simulink model "BimanualCarvingModifiedOldEMG"  (R2013a)
settings: Solver=ode4  SolverMode=SingleTasking  StartTime=0.0  StopTime=inf  FixedStep=0.0005  RelTol=1e-3
StartFcn:
  |  warndlg('Dexterit-E models cannot run under simulation. Please compile your model and run it from within Dexterit-E.');set_param(bdroot,'SimulationCommand','stop')
model workspace (MAT data in the model file):
  BKIN_STEP_TIME = 0.0005
  col_x = 1
  col_y = 2
  WIDTH = 3
  HEIGHT = 4
  TARGET_COL = 1
  LOAD = 2
  TRAJ_DURATION_COL = 3
  MAX_LOAD = 2
  FORCE_ON = 1
  HAND_RADIUS = 6
  REST_COL = 4
  TRAINING_COL = 5
  HAND_COLOR = 5
  TARGET_STROKE = 8
  TARGET_RADIUS = 9
  xMaxCursor = 15
  yMaxCursor = 16
  TARGET_COLOR = 7
  START_X = 10
  START_Y = 11
  STIFFNESS_MATERIAL = 3
  MATERIAL_MASS = 4
  MATERIAL_DAMPING = 5
  STIFFNESS_HANDS = 6
  MATERIAL_GOAL_COLOR = 12
  SCALE_VIBRATION = 7
  STONE_WIDTH = 6
  MATERIAL_DUCTILITY = 8
  TARG_COLOR = 1
  TEXT_COLOR = 13
  TEXTBOX_WIDTH = 14
  TEXTBOX_HEIGHT = 15
  ROTATION = 16
  LABEL_TEXT = 17
  LABEL_COLOR = 18
  LABEL_HEIGHT = 19
  ADVANCE_EMG_PLACEMENT = 2
  ADVANCE_EMG_MAX = 3
  EMG_ADVANCE_BUTTON = 1
  EMG_MVC_BUTTON = 2
  START_TRIAL = 3
  END_TRIAL = 4
  MUSC_NUM = 2
  HAND_DISTANCE = 3
  SYN_NUM = 4
undefined symbols (not defined in the file or in its folder): slselsubs
libraries: xpclib x9, simulink x6, General x3, KINARM_loads x2, Video x2, KINARM_IO x1, KINARM_EP_loads x1
(part 5 of 6)

== matlab function BimanualCarvingModifiedOldEMG/Draw_Material/MATLAB Function ==
  data: target input; VCODE output; state_in input; target_type input; opacity_in input; target_display input; x_index input; y_index input; num_states input; stateindices input; target_labels input; KINData input; MaterialPos input; trial_state input
function VCODE = fcn(target, state_in, target_type, opacity_in, target_display, x_index, y_index, num_states, stateindices, target_labels, KINData, MaterialPos, trial_state)

% stateindices should follow this order (depending on target-type):
% 1: fill colour
% 2: stroke colour
% 3: stroke width
% 4: major radius / radius / start point (line)
% 5: minor radius / end point (line)
% 6: orientation angle



% VCODEs are length 70. All units in a VCODE should be SI, e.g. (m) and (rad). Elements in a VCODE are defined as follows:
%
% For all target types:
%  1: target type
%       1 - circle
%       2 - ellipse
%       3 - rectangle
%       4 - line
%       5 - triangle
%       11 - circle with label
%       12 - ellipse with label
%       13 - rectangle with label
%       14 - line with label
%       15 - triangle with label
%  2: target on/off status and target display (which display target will appear on)
%		0 - off
%		1 - on, appearing on both subject and operator displays
%       2 - on, appearing on subject display only
%       3 - on, appearing on operator display only
%  3: x position (m)
%  4: y position (m)
%  5: fill colour (RRGGBB) or texture index
%  6: stroke colour (RRGGBB) or texture index
%  7: stroke width
%  8: reserved for target background ID
%  9: opacity
%
% For circles:
%  10: radius (m)
%
% For ellipses:
%  10: major radius (m)
%  11: minor radius (m)
%  12: orientation of major axis (rad)
%
% For rectangles:
%  10: length (m)
%  11: height (m)
%  12: orientation (rad) (relative to x, y already shown)
%
% For lines:
%  10: endpoint x-axis coordinate relative to start point (m)
%  11: endpoint y-axis coordinate relative to start point (m)
%
% For triangles:
%  10: length (m)
%  11: height (m)
%  12: offset of peak from midpoint of length (m)
%  13: orientation (rad)
%
% For all labelled target types:
%  14: reserved
%  15-64: label characters (indexes in ISO 8859-1 character set)
%  65: label colour (0xRRGGBB), opacity is set by the vcode's opacity (9).
%  66: label height (m)
%  67: reserved
%  68: reserved
%  69: reserved
%  70: reserved

num_targets = size(MaterialPos,2)-1;

% NOTE: we assume that the STATE and/or OPACITY inputs are vectors. 

% If the length of the input STATE is not the same as the number of targets then make STATE a column vector of the same length as 
% the TARGET input, using the first STATE (i.e. all targets get the same state)
if num_targets == length(state_in)
	state = reshape(state_in, num_targets, 1);
else
	state = state_in(1) * ones(num_targets, 1);
end


% If the length of the input OPACITY is not the same as the number of targets then make OPACITY a column vector of the same length as
% the TARGET input, using the first OPACITY (i.e. all targets get the same opacity)
if num_targets == length(opacity_in)
	opacity = reshape(opacity_in, num_targets, 1);
else
	opacity = opacity_in(1) * ones(num_targets, 1);
end


% Clamping the opacity to [0, 100].
opacity = min(opacity, 100);
opacity = max(opacity, 0);

VCODE = zeros(num_targets, 70);

% Set the target type. Targets with labels have type codes 10 greater than their unlabelled counterparts.
VCODE(:, 1) = target_type + 10;
VCODE(:, 2) = target_display;

VCODE(:, 5) = colourshift(target(1, stateindices(state(1), 1)));
VCODE(:, 6) = colourshift(target(1, stateindices(state(1), 1)));

% Set the opacity value
VCODE(:, 9) = opacity_in(1);
% Target only visible during tracking in trial_state==2
%{
if trial_state==0
    VCODE(:, 5) = colourshift(1000000000);
    VCODE(:, 6) = colourshift(1000000000);
    VCODE(:, 9) = 0;
end
%}

% Stroke width
VCODE(:, 7) = target(1, stateindices(state(1), 3))*0.01;

VCODE(:, 3) = MaterialPos(1,1:end-1)';  % x position (m)
VCODE(:, 4) = MaterialPos(2,1:end-1)';  % y position (m)

VCODE(:, 10) = MaterialPos(1,2:end)'-VCODE(:,3);  % line endpoint in x axis, relative to start (m)
VCODE(:, 11) = MaterialPos(2,2:end)'-VCODE(:,4);  % line endpoint in y axis, relative to start (m)

%{
persistent TargetIndex;
if isempty(TargetIndex), TargetIndex = 1; end
% Set the hand position.
if TargetIndex<=length(xMaterial)
    % Initially draw the whole material from left to right
    % Line beginning
    VCODE(:, 3) = xMaterial(TargetIndex);  % x position (m)
    VCODE(:, 4) = yMaterial(TargetIndex);  % y position (m)
    
    % Line endpoint
    VCODE(:, 10) = xMaterial(TargetIndex+1)-VCODE(:,3);  % line endpoint in x axis, relative to start (m)
    VCODE(:, 11) = yMaterial(TargetIndex+1)-VCODE(:,4);  % line endpoint in y axis, relative to start (m)
else
    % After material is all drawn, update only the changing section
    % Line beginning
    VCODE(:, 3) = xMaterial(MaterialUpdateInd1);  % x position (m)
    VCODE(:, 4) = yMaterial(MaterialUpdateInd1);  % y position (m)
    
    % Line endpoint
    VCODE(:, 10) = xMaterial(MaterialUpdateInd2)-VCODE(:,3);  % line endpoint in x axis, relative to start (m)
    VCODE(:, 11) = yMaterial(MaterialUpdateInd2)-VCODE(:,4);  % line endpoint in y axis, relative to start (m)
end


TargetIndex = min(length(xMaterial)+5,TargetIndex+1);
%}
%{
for ii = 1:num_targets
	% Set the target on/off state. If the state input is 0, the target is off. Users of the VCODE should respect this
	% as an indication that the rest of the VCODE will be uninitialized.
	if (state(ii) <= 0) || (state(ii) > num_states)
		VCODE(ii, 2) = 0;  % target is off
	else
		VCODE(ii, 2) = target_display;  % Default is that target is on; target displays as specified by block mask
	end

	fill_colour_col = stateindices(state(ii), 1);
	stroke_colour_col = stateindices(state(ii), 2);
	stroke_width_col = stateindices(state(ii), 3);
	
	% Set the fill colour. Fill colour currently comes from the GUI in RRRGGGBBB format.
	%{
    if fill_colour_col == 0
		VCODE(ii, 5) = -2^31;
	elseif target(fill_colour_col) < 0
		VCODE(ii, 5) = target(ii, fill_colour_col);
	else
		VCODE(ii, 5) = colourshift(target(ii, fill_colour_col));
    end
    %}
    VCODE(ii,5) = colourshift(1000000000);
	
	% Set the stroke colour. Stroke colour currently comes from the GUI in RRRGGGBBB format.
    if trial_state==1
        if stroke_colour_col == 0
            VCODE(ii, 6) = -2^31;
        elseif target(stroke_colour_col) < 0
            VCODE(ii, 6) = target(ii, stroke_colour_col);
        else
            VCODE(ii, 6) = colourshift( target(ii, stroke_colour_col) );
        end
    else
        % CIRCLE APPEARS ONLY DURING TASK
        VCODE(ii, 6) = colourshift(1000000000);
    end

	% Set the stroke width. if target table index for stroke width is zero, then the stroke width is undefined
	if stroke_width_col == 0
		VCODE(ii, 7) = 0;                   % if stroke width column is 0, then stroke width is 0
	elseif stroke_width_col < 0
		VCODE(ii, 7) = 0.001;               % if stroke width column is -ve, then a 1mm default is chosen
	else
		VCODE(ii, 7) = target(ii, stroke_width_col) * 0.01;  % if stroke width column is +ve, convert width from (cm) in target table to (m)
    end

	% Set the opacity value
	VCODE(ii, 9) = opacity(ii);

	% Set attributes specific to each target type. In the process, note the first state vector column used for label information.
	label_index = 1;

	% Set attributes specific to each target type.
	if target_type == 1

		% Handle circle target:
		radius_col = stateindices(state(ii), 4);
		VCODE(ii, 10)=target(ii, radius_col);  % radius (in m)
	    label_index = 5;

	elseif target_type == 2 || target_type == 3

	    % Handle ellipse or rectangle target:
		major_col = stateindices(state(ii), 4);
		minor_col = stateindices(state(ii), 5);
		orientation_col = stateindices(state(ii), 6);
		
		VCODE(ii, 10) = target(ii, major_col) * 0.01;  % major radius (convert from (cm) in target table to (m))
		VCODE(ii, 11) = target(ii, minor_col) * 0.01;  % minor radius (convert from (cm) in target table to (m))
		if orientation_col == 0
			VCODE(ii, 12) = 0;  % if orientation column is 0, set orientation to 0 rad
		else
			VCODE(ii, 12) = mod(target(ii, orientation_col), 360) * pi / 180.0;  % orientation (convert from (degrees) in target table to (rad))
		end
	    label_index = 7;
	
	elseif target_type == 4

		% Handle line target:
		%xendpoint_col = stateindices(state(ii), 4);
		%yendpoint_col = stateindices(state(ii), 5);
		VCODE(ii, 10) = 0;  % line endpoint in x axis, relative to start (m)
		VCODE(ii, 11) = stateindices(state(ii), 1);  % line endpoint in y axis, relative to start (taken from Target Table)
	    label_index = 6;

	elseif target_type == 5

		% Handle triangle target:
		length_col = stateindices(state(ii), 4);
		height_col = stateindices(state(ii), 5);
		offset_col = stateindices(state(ii), 6);
		orientation_col = stateindices(state(ii), 7);

		VCODE(ii, 10) = target(ii, length_col) * 0.01;  % length (convert from (cm) in target table to (m))

		% If the height column is set to 0 then the triangle is automatically made equilateral, with the base length used as length
		% for all sides. If the height column is non-zero, separate values for height and peak offset are taken from the target table.
		if height_col == 0
			VCODE(ii, 11) = sin(pi / 3.0) * VCODE(ii, 10);  % height for equilateral triangle
			VCODE(ii, 12) = 0;                          % peak offset for equilateral triangle
		else
			VCODE(ii, 11) = target(ii, height_col) * 0.01;  % height (convert from (cm) in target table to (m))
			VCODE(ii, 12) = target(ii, offset_col) * 0.01;  % peak offset (convert from (cm) in target table to (m))
		end

		if orientation_col == 0
			VCODE(ii, 13) = 0;  % if orientation column is 0, set orientation to 0 rad
		else
			VCODE(ii, 13) = mod(target(ii, orientation_col), 360) * pi / 180.0;  % orientation (convert from (degrees) in target table to (rad))
		end
	    label_index = 8;
		
	end
	
	% Copy the label characters to the VCODE.
	for jj = 1:50
		VCODE(ii, jj + 14) = target_labels( target( ii, stateindices(state(ii), label_index) ), jj );
	end

	% Set the label colour. Like other colours, label colour comes from the GUI in RRRGGGBBB format and is converted to a 32-bit
	% 0xRRGGBB value here. If the target column table index for the colour is 0, the label is transparent.
	if stateindices(state(ii), label_index + 1) == 0
		VCODE(ii, 65) = -2^31;
	elseif target( ii, stateindices(state(ii), label_index + 1) ) < 0
		VCODE(ii, 65) = target( ii, stateindices(state(ii), label_index + 1) );
	else
		VCODE(ii, 65) = colourshift( target( ii, stateindices(state(ii), label_index + 1) ) );
	end

	% Set the label height. Label height is converted from (cm) in the target table to (m).
	VCODE(ii, 66) = target( ii, stateindices(state, label_index + 2) ) * 0.01;


	
end
%}
% The colourshift function converts an "RRRGGGBBB" colour value to RRGBB (as an uint32).
function RRGGBBAA = colourshift(RRRGGGBBB)

%this is "no fill"
if RRRGGGBBB == 1000000000
    RRGGBBAA = cast(16777216, 'uint32'); %hex 0x1000000
    return; 
end

blue = cast(mod(RRRGGGBBB, 1000), 'uint32');
green = cast(mod(RRRGGGBBB - blue, 1000000) / 1000, 'uint32');
red = cast((RRRGGGBBB - (green * 1000) - blue) / 1000000, 'uint32');

RRGGBBAA = bitshift(red, 16) + bitshift(green, 8) + blue;

== matlab function BimanualCarvingModifiedOldEMG/Draw_Start/MATLAB Function ==
  data: target input; VCODE output; state_in input; target_type input; opacity_in input; target_display input; x_index input; y_index input; num_states input; stateindices input; target_labels input; KINData input; xStart input; yStart input; HandDistance input; trial_state input
function VCODE = fcn(target, state_in, target_type, opacity_in, target_display, x_index, y_index, num_states, stateindices, target_labels, KINData, xStart, yStart, HandDistance, trial_state)

% stateindices should follow this order (depending on target-type):
% 1: fill colour
% 2: stroke colour
% 3: stroke width
% 4: major radius / radius / start point (line)
% 5: minor radius / end point (line)
% 6: orientation angle



% VCODEs are length 70. All units in a VCODE should be SI, e.g. (m) and (rad). Elements in a VCODE are defined as follows:
%
% For all target types:
%  1: target type
%       1 - circle
%       2 - ellipse
%       3 - rectangle
%       4 - line
%       5 - triangle
%       11 - circle with label
%       12 - ellipse with label
%       13 - rectangle with label
%       14 - line with label
%       15 - triangle with label
%  2: target on/off status and target display (which display target will appear on)
%		0 - off
%		1 - on, appearing on both subject and operator displays
%       2 - on, appearing on subject display only
%       3 - on, appearing on operator display only
%  3: x position (m)
%  4: y position (m)
%  5: fill colour (RRGGBB) or texture index
%  6: stroke colour (RRGGBB) or texture index
%  7: stroke width
%  8: reserved for target background ID
%  9: opacity
%
% For circles:
%  10: radius (m)
%
% For ellipses:
%  10: major radius (m)
%  11: minor radius (m)
%  12: orientation of major axis (rad)
%
% For rectangles:
%  10: length (m)
%  11: height (m)
%  12: orientation (rad) (relative to x, y already shown)
%
% For lines:
%  10: endpoint x-axis coordinate relative to start point (m)
%  11: endpoint y-axis coordinate relative to start point (m)
%
% For triangles:
%  10: length (m)
%  11: height (m)
%  12: offset of peak from midpoint of length (m)
%  13: orientation (rad)
%
% For all labelled target types:
%  14: reserved
%  15-64: label characters (indexes in ISO 8859-1 character set)
%  65: label colour (0xRRGGBB), opacity is set by the vcode's opacity (9).
%  66: label height (m)
%  67: reserved
%  68: reserved
%  69: reserved
%  70: reserved

num_targets = 2;

% NOTE: we assume that the STATE and/or OPACITY inputs are vectors. 

% If the length of the input STATE is not the same as the number of targets then make STATE a column vector of the same length as 
% the TARGET input, using the first STATE (i.e. all targets get the same state)
if num_targets == length(state_in)
	state = reshape(state_in, num_targets, 1);
else
	state = state_in(1) * ones(num_targets, 1);
end


% If the length of the input OPACITY is not the same as the number of targets then make OPACITY a column vector of the same length as
% the TARGET input, using the first OPACITY (i.e. all targets get the same opacity)
if num_targets == length(opacity_in)
	opacity = reshape(opacity_in, num_targets, 1);
else
	opacity = opacity_in(1) * ones(num_targets, 1);
end


% Clamping the opacity to [0, 100].
opacity = min(opacity, 100);
opacity = max(opacity, 0);

VCODE = zeros(num_targets, 70);

% Set the target type. Targets with labels have type codes 10 greater than their unlabelled counterparts.
VCODE(:, 1) = target_type + 10;

% Set the hand position.
VCODE(1, 3) = xStart+HandDistance/2;  % x position (m)
VCODE(1, 4) = yStart;  % y position (m)
VCODE(2, 3) = xStart-HandDistance/2;  % x position (m)
VCODE(2, 4) = yStart;  % y position (m)

for ii = 1:num_targets
	% Set the target on/off state. If the state input is 0, the target is off. Users of the VCODE should respect this
	% as an indication that the rest of the VCODE will be uninitialized.
    
	if (state(1) <= 0) || (state(1) > num_states)
		VCODE(ii, 2) = 0;  % target is off
	else
		VCODE(ii, 2) = target_display;  % Default is that target is on; target displays as specified by block mask
    end
    

	fill_colour_col = stateindices(state(1), 1);
	stroke_colour_col = stateindices(state(1), 2);
	stroke_width_col = stateindices(state(1), 3);
	
	% Set the fill colour. Fill colour currently comes from the GUI in RRRGGGBBB format.
	%{
    if fill_colour_col == 0
		VCODE(ii, 5) = -2^31;
	elseif target(fill_colour_col) < 0
		VCODE(ii, 5) = target(ii, fill_colour_col);
	else
		VCODE(ii, 5) = colourshift(target(ii, fill_colour_col));
    end
    %}
    VCODE(ii,5) = colourshift(1000000000);
	
	% Set the stroke colour. Stroke colour currently comes from the GUI in RRRGGGBBB format.
	if stroke_colour_col == 0
		VCODE(ii, 6) = -2^31;
	elseif target(stroke_colour_col) < 0
		VCODE(ii, 6) = target(1, stroke_colour_col);
	else
		VCODE(ii, 6) = colourshift( target(1, stroke_colour_col) );
    end
    if trial_state~=0
        VCODE(ii,5) = colourshift(1000000000);
    end

	% Set the stroke width. if target table index for stroke width is zero, then the stroke width is undefined
	if stroke_width_col == 0
		VCODE(ii, 7) = 0;                   % if stroke width column is 0, then stroke width is 0
	elseif stroke_width_col < 0
		VCODE(ii, 7) = 0.001;               % if stroke width column is -ve, then a 1mm default is chosen
	else
		VCODE(ii, 7) = target(1, stroke_width_col) * 0.01 * 3;  % if stroke width column is +ve, convert width from (cm) in target table to (m)
    end
    if trial_state==1
        VCODE(ii,7) = 0;
    end

	% Set the opacity value
    VCODE(ii, 9) = 100;

	% Set attributes specific to each target type. In the process, note the first state vector column used for label information.
	label_index = 1;

	% Set attributes specific to each target type.
	if target_type == 1

		% Handle circle target:
		radius_col = stateindices(state(1), 4);
		VCODE(ii, 10)=target(1, radius_col);  % radius (in m)
	    label_index = 5;

	elseif target_type == 2 || target_type == 3

	    % Handle ellipse or rectangle target:
		major_col = stateindices(state(ii), 4);
		minor_col = stateindices(state(ii), 5);
		orientation_col = stateindices(state(ii), 6);
		
		VCODE(ii, 10) = target(ii, major_col) * 0.01;  % major radius (convert from (cm) in target table to (m))
		VCODE(ii, 11) = target(ii, minor_col) * 0.01;  % minor radius (convert from (cm) in target table to (m))
		if orientation_col == 0
			VCODE(ii, 12) = 0;  % if orientation column is 0, set orientation to 0 rad
		else
			VCODE(ii, 12) = mod(target(ii, orientation_col), 360) * pi / 180.0;  % orientation (convert from (degrees) in target table to (rad))
		end
	    label_index = 7;
	
	elseif target_type == 4

		% Handle line target:
		%xendpoint_col = stateindices(state(ii), 4);
		%yendpoint_col = stateindices(state(ii), 5);
		VCODE(ii, 10) = 0;  % line endpoint in x axis, relative to start (m)
		VCODE(ii, 11) = stateindices(state(ii), 1);  % line endpoint in y axis, relative to start (taken from Target Table)
	    label_index = 6;

	elseif target_type == 5

		% Handle triangle target:
		length_col = stateindices(state(ii), 4);
		height_col = stateindices(state(ii), 5);
		offset_col = stateindices(state(ii), 6);
		orientation_col = stateindices(state(ii), 7);

		VCODE(ii, 10) = target(ii, length_col) * 0.01;  % length (convert from (cm) in target table to (m))

		% If the height column is set to 0 then the triangle is automatically made equilateral, with the base length used as length
		% for all sides. If the height column is non-zero, separate values for height and peak offset are taken from the target table.
		if height_col == 0
			VCODE(ii, 11) = sin(pi / 3.0) * VCODE(ii, 10);  % height for equilateral triangle
			VCODE(ii, 12) = 0;                          % peak offset for equilateral triangle
		else
			VCODE(ii, 11) = target(ii, height_col) * 0.01;  % height (convert from (cm) in target table to (m))
			VCODE(ii, 12) = target(ii, offset_col) * 0.01;  % peak offset (convert from (cm) in target table to (m))
		end

		if orientation_col == 0
			VCODE(ii, 13) = 0;  % if orientation column is 0, set orientation to 0 rad
		else
			VCODE(ii, 13) = mod(target(ii, orientation_col), 360) * pi / 180.0;  % orientation (convert from (degrees) in target table to (rad))
		end
	    label_index = 8;
		
	end
	%{
	% Copy the label characters to the VCODE.
	for jj = 1:50
		VCODE(ii, jj + 14) = target_labels( target( ii, stateindices(state(ii), label_index) ), jj );
	end

	% Set the label colour. Like other colours, label colour comes from the GUI in RRRGGGBBB format and is converted to a 32-bit
	% 0xRRGGBB value here. If the target column table index for the colour is 0, the label is transparent.
	if stateindices(state(ii), label_index + 1) == 0
		VCODE(ii, 65) = -2^31;
	elseif target( ii, stateindices(state(ii), label_index + 1) ) < 0
		VCODE(ii, 65) = target( ii, stateindices(state(ii), label_index + 1) );
	else
		VCODE(ii, 65) = colourshift( target( ii, stateindices(state(ii), label_index + 1) ) );
	end

	% Set the label height. Label height is converted from (cm) in the target table to (m).
	VCODE(ii, 66) = target( ii, stateindices(state, label_index + 2) ) * 0.01;
    %}

	
end

% The colourshift function converts an "RRRGGGBBB" colour value to RRGBB (as an uint32).
function RRGGBBAA = colourshift(RRRGGGBBB)

%this is "no fill"
if RRRGGGBBB == 1000000000
    RRGGBBAA = cast(16777216, 'uint32'); %hex 0x1000000
    return; 
end

blue = cast(mod(RRRGGGBBB, 1000), 'uint32');
green = cast(mod(RRRGGGBBB - blue, 1000000) / 1000, 'uint32');
red = cast((RRRGGGBBB - (green * 1000) - blue) / 1000000, 'uint32');

RRGGBBAA = bitshift(red, 16) + bitshift(green, 8) + blue;

== matlab function BimanualCarvingModifiedOldEMG/Draw_MaterialTarget/MATLAB Function ==
  data: target input; VCODE output; state_in input; target_type input; opacity_in input; target_display input; x_index input; y_index input; num_states input; stateindices input; target_labels input; KINData input; MaterialPos input; trial_state input
function VCODE = fcn(target, state_in, target_type, opacity_in, target_display, x_index, y_index, num_states, stateindices, target_labels, KINData, MaterialPos, trial_state)

% stateindices should follow this order (depending on target-type):
% 1: fill colour
% 2: stroke colour
% 3: stroke width
% 4: major radius / radius / start point (line)
% 5: minor radius / end point (line)
% 6: orientation angle



% VCODEs are length 70. All units in a VCODE should be SI, e.g. (m) and (rad). Elements in a VCODE are defined as follows:
%
% For all target types:
%  1: target type
%       1 - circle
%       2 - ellipse
%       3 - rectangle
%       4 - line
%       5 - triangle
%       11 - circle with label
%       12 - ellipse with label
%       13 - rectangle with label
%       14 - line with label
%       15 - triangle with label
%  2: target on/off status and target display (which display target will appear on)
%		0 - off
%		1 - on, appearing on both subject and operator displays
%       2 - on, appearing on subject display only
%       3 - on, appearing on operator display only
%  3: x position (m)
%  4: y position (m)
%  5: fill colour (RRGGBB) or texture index
%  6: stroke colour (RRGGBB) or texture index
%  7: stroke width
%  8: reserved for target background ID
%  9: opacity
%
% For circles:
%  10: radius (m)
%
% For ellipses:
%  10: major radius (m)
%  11: minor radius (m)
%  12: orientation of major axis (rad)
%
% For rectangles:
%  10: length (m)
%  11: height (m)
%  12: orientation (rad) (relative to x, y already shown)
%
% For lines:
%  10: endpoint x-axis coordinate relative to start point (m)
%  11: endpoint y-axis coordinate relative to start point (m)
%
% For triangles:
%  10: length (m)
%  11: height (m)
%  12: offset of peak from midpoint of length (m)
%  13: orientation (rad)
%
% For all labelled target types:
%  14: reserved
%  15-64: label characters (indexes in ISO 8859-1 character set)
%  65: label colour (0xRRGGBB), opacity is set by the vcode's opacity (9).
%  66: label height (m)
%  67: reserved
%  68: reserved
%  69: reserved
%  70: reserved

num_targets = size(MaterialPos,2)-1;

% NOTE: we assume that the STATE and/or OPACITY inputs are vectors. 

% If the length of the input STATE is not the same as the number of targets then make STATE a column vector of the same length as 
% the TARGET input, using the first STATE (i.e. all targets get the same state)
if num_targets == length(state_in)
	state = reshape(state_in, num_targets, 1);
else
	state = state_in(1) * ones(num_targets, 1);
end


% If the length of the input OPACITY is not the same as the number of targets then make OPACITY a column vector of the same length as
% the TARGET input, using the first OPACITY (i.e. all targets get the same opacity)
if num_targets == length(opacity_in)
	opacity = reshape(opacity_in, num_targets, 1);
else
	opacity = opacity_in(1) * ones(num_targets, 1);
end


% Clamping the opacity to [0, 100].
opacity = min(opacity, 100);
opacity = max(opacity, 0);

VCODE = zeros(num_targets, 70);

% Set the target type. Targets with labels have type codes 10 greater than their unlabelled counterparts.
VCODE(:, 1) = target_type + 10;
VCODE(:, 2) = target_display;

VCODE(:, 5) = colourshift(target(1, stateindices(state(1), 1)));
VCODE(:, 6) = colourshift(target(1, stateindices(state(1), 1)));

% Set the opacity value
VCODE(:, 9) = opacity_in(1);
% Target only visible during tracking in trial_state==2
%{
if trial_state==0
    VCODE(:, 5) = colourshift(1000000000);
    VCODE(:, 6) = colourshift(1000000000);
    VCODE(:, 9) = 0;
end
%}

% Stroke width
VCODE(:, 7) = target(1, stateindices(state(1), 3))*0.01;

VCODE(:, 3) = MaterialPos(1,1:end-1)';  % x position (m)
VCODE(:, 4) = MaterialPos(2,1:end-1)';  % y position (m)

VCODE(:, 10) = MaterialPos(1,2:end)'-VCODE(:,3);  % line endpoint in x axis, relative to start (m)
VCODE(:, 11) = MaterialPos(2,2:end)'-VCODE(:,4);  % line endpoint in y axis, relative to start (m)

%{
persistent TargetIndex;
if isempty(TargetIndex), TargetIndex = 1; end
% Set the hand position.
if TargetIndex<=length(xMaterial)
    % Initially draw the whole material from left to right
    % Line beginning
    VCODE(:, 3) = xMaterial(TargetIndex);  % x position (m)
    VCODE(:, 4) = yMaterial(TargetIndex);  % y position (m)
    
    % Line endpoint
    VCODE(:, 10) = xMaterial(TargetIndex+1)-VCODE(:,3);  % line endpoint in x axis, relative to start (m)
    VCODE(:, 11) = yMaterial(TargetIndex+1)-VCODE(:,4);  % line endpoint in y axis, relative to start (m)
else
    % After material is all drawn, update only the changing section
    % Line beginning
    VCODE(:, 3) = xMaterial(MaterialUpdateInd1);  % x position (m)
    VCODE(:, 4) = yMaterial(MaterialUpdateInd1);  % y position (m)
    
    % Line endpoint
    VCODE(:, 10) = xMaterial(MaterialUpdateInd2)-VCODE(:,3);  % line endpoint in x axis, relative to start (m)
    VCODE(:, 11) = yMaterial(MaterialUpdateInd2)-VCODE(:,4);  % line endpoint in y axis, relative to start (m)
end


TargetIndex = min(length(xMaterial)+5,TargetIndex+1);
%}
%{
for ii = 1:num_targets
	% Set the target on/off state. If the state input is 0, the target is off. Users of the VCODE should respect this
	% as an indication that the rest of the VCODE will be uninitialized.
	if (state(ii) <= 0) || (state(ii) > num_states)
		VCODE(ii, 2) = 0;  % target is off
	else
		VCODE(ii, 2) = target_display;  % Default is that target is on; target displays as specified by block mask
	end

	fill_colour_col = stateindices(state(ii), 1);
	stroke_colour_col = stateindices(state(ii), 2);
	stroke_width_col = stateindices(state(ii), 3);
	
	% Set the fill colour. Fill colour currently comes from the GUI in RRRGGGBBB format.
	%{
    if fill_colour_col == 0
		VCODE(ii, 5) = -2^31;
	elseif target(fill_colour_col) < 0
		VCODE(ii, 5) = target(ii, fill_colour_col);
	else
		VCODE(ii, 5) = colourshift(target(ii, fill_colour_col));
    end
    %}
    VCODE(ii,5) = colourshift(1000000000);
	
	% Set the stroke colour. Stroke colour currently comes from the GUI in RRRGGGBBB format.
    if trial_state==1
        if stroke_colour_col == 0
            VCODE(ii, 6) = -2^31;
        elseif target(stroke_colour_col) < 0
            VCODE(ii, 6) = target(ii, stroke_colour_col);
        else
            VCODE(ii, 6) = colourshift( target(ii, stroke_colour_col) );
        end
    else
        % CIRCLE APPEARS ONLY DURING TASK
        VCODE(ii, 6) = colourshift(1000000000);
    end

	% Set the stroke width. if target table index for stroke width is zero, then the stroke width is undefined
	if stroke_width_col == 0
		VCODE(ii, 7) = 0;                   % if stroke width column is 0, then stroke width is 0
	elseif stroke_width_col < 0
		VCODE(ii, 7) = 0.001;               % if stroke width column is -ve, then a 1mm default is chosen
	else
		VCODE(ii, 7) = target(ii, stroke_width_col) * 0.01;  % if stroke width column is +ve, convert width from (cm) in target table to (m)
    end

	% Set the opacity value
	VCODE(ii, 9) = opacity(ii);

	% Set attributes specific to each target type. In the process, note the first state vector column used for label information.
	label_index = 1;

	% Set attributes specific to each target type.
	if target_type == 1

		% Handle circle target:
		radius_col = stateindices(state(ii), 4);
		VCODE(ii, 10)=target(ii, radius_col);  % radius (in m)
	    label_index = 5;

	elseif target_type == 2 || target_type == 3

	    % Handle ellipse or rectangle target:
		major_col = stateindices(state(ii), 4);
		minor_col = stateindices(state(ii), 5);
		orientation_col = stateindices(state(ii), 6);
		
		VCODE(ii, 10) = target(ii, major_col) * 0.01;  % major radius (convert from (cm) in target table to (m))
		VCODE(ii, 11) = target(ii, minor_col) * 0.01;  % minor radius (convert from (cm) in target table to (m))
		if orientation_col == 0
			VCODE(ii, 12) = 0;  % if orientation column is 0, set orientation to 0 rad
		else
			VCODE(ii, 12) = mod(target(ii, orientation_col), 360) * pi / 180.0;  % orientation (convert from (degrees) in target table to (rad))
		end
	    label_index = 7;
	
	elseif target_type == 4

		% Handle line target:
		%xendpoint_col = stateindices(state(ii), 4);
		%yendpoint_col = stateindices(state(ii), 5);
		VCODE(ii, 10) = 0;  % line endpoint in x axis, relative to start (m)
		VCODE(ii, 11) = stateindices(state(ii), 1);  % line endpoint in y axis, relative to start (taken from Target Table)
	    label_index = 6;

	elseif target_type == 5

		% Handle triangle target:
		length_col = stateindices(state(ii), 4);
		height_col = stateindices(state(ii), 5);
		offset_col = stateindices(state(ii), 6);
		orientation_col = stateindices(state(ii), 7);

		VCODE(ii, 10) = target(ii, length_col) * 0.01;  % length (convert from (cm) in target table to (m))

		% If the height column is set to 0 then the triangle is automatically made equilateral, with the base length used as length
		% for all sides. If the height column is non-zero, separate values for height and peak offset are taken from the target table.
		if height_col == 0
			VCODE(ii, 11) = sin(pi / 3.0) * VCODE(ii, 10);  % height for equilateral triangle
			VCODE(ii, 12) = 0;                          % peak offset for equilateral triangle
		else
			VCODE(ii, 11) = target(ii, height_col) * 0.01;  % height (convert from (cm) in target table to (m))
			VCODE(ii, 12) = target(ii, offset_col) * 0.01;  % peak offset (convert from (cm) in target table to (m))
		end

		if orientation_col == 0
			VCODE(ii, 13) = 0;  % if orientation column is 0, set orientation to 0 rad
		else
			VCODE(ii, 13) = mod(target(ii, orientation_col), 360) * pi / 180.0;  % orientation (convert from (degrees) in target table to (rad))
		end
	    label_index = 8;
		
	end
	
	% Copy the label characters to the VCODE.
	for jj = 1:50
		VCODE(ii, jj + 14) = target_labels( target( ii, stateindices(state(ii), label_index) ), jj );
	end

	% Set the label colour. Like other colours, label colour comes from the GUI in RRRGGGBBB format and is converted to a 32-bit
	% 0xRRGGBB value here. If the target column table index for the colour is 0, the label is transparent.
	if stateindices(state(ii), label_index + 1) == 0
		VCODE(ii, 65) = -2^31;
	elseif target( ii, stateindices(state(ii), label_index + 1) ) < 0
		VCODE(ii, 65) = target( ii, stateindices(state(ii), label_index + 1) );
	else
		VCODE(ii, 65) = colourshift( target( ii, stateindices(state(ii), label_index + 1) ) );
	end

	% Set the label height. Label height is converted from (cm) in the target table to (m).
	VCODE(ii, 66) = target( ii, stateindices(state, label_index + 2) ) * 0.01;


	
end
%}
% The colourshift function converts an "RRRGGGBBB" colour value to RRGBB (as an uint32).
function RRGGBBAA = colourshift(RRRGGGBBB)

%this is "no fill"
if RRRGGGBBB == 1000000000
    RRGGBBAA = cast(16777216, 'uint32'); %hex 0x1000000
    return; 
end

blue = cast(mod(RRRGGGBBB, 1000), 'uint32');
green = cast(mod(RRRGGGBBB - blue, 1000000) / 1000, 'uint32');
red = cast((RRRGGGBBB - (green * 1000) - blue) / 1000000, 'uint32');

RRGGBBAA = bitshift(red, 16) + bitshift(green, 8) + blue;

== matlab function BimanualCarvingModifiedOldEMG/Parameter_columns/MATLAB Function ==
  data: target input; VCODE output; state_in input; target_type input; opacity_in input; target_display input; x_index input; y_index input; num_states input; stateindices input; target_labels input
function VCODE = fcn(target, state_in, target_type, opacity_in, target_display, x_index, y_index, num_states, stateindices, target_labels)

VCODE = zeros(1,70);
% SIMPLY ASSIGN TOOL LENGTH AND WIDTH TO OUTPUT, NOT REAL VCODE!!
VCODE(1,1) = target(1,stateindices(1,1)); % tool width (m)
VCODE(1,2) = target(1,stateindices(1,2)); % tool length (m)
VCODE(1,3) = target(1,stateindices(1,3)); % frame inner width (m)
VCODE(1,4) = target(1,stateindices(1,4)); % frame outer width (m)
VCODE(1,5) = target(1,stateindices(1,5)); % force on?
VCODE(1,6) = target(1,stateindices(1,6)); % start radius (m)
VCODE(1,7) = target(1,stateindices(1,7)); % end radius (m)
%{
% stateindices should follow this order (depending on target-type):
% 1: fill colour
% 2: stroke colour
% 3: stroke width
% 4: major radius / radius / start point (line)
% 5: minor radius / end point (line)
% 6: orientation angle



% VCODEs are length 70. All units in a VCODE should be SI, e.g. (m) and (rad). Elements in a VCODE are defined as follows:
%
% For all target types:
%  1: target type
%       1 - circle
%       2 - ellipse
%       3 - rectangle
%       4 - line
%       5 - triangle
%       11 - circle with label
%       12 - ellipse with label
%       13 - rectangle with label
%       14 - line with label
%       15 - triangle with label
%  2: target on/off status and target display (which display target will appear on)
%		0 - off
%		1 - on, appearing on both subject and operator displays
%       2 - on, appearing on subject display only
%       3 - on, appearing on operator display only
%  3: x position (m)
%  4: y position (m)
%  5: fill colour (RRGGBB) or texture index
%  6: stroke colour (RRGGBB) or texture index
%  7: stroke width
%  8: reserved for target background ID
%  9: opacity
%
% For circles:
%  10: radius (m)
%
% For ellipses:
%  10: major radius (m)
%  11: minor radius (m)
%  12: orientation of major axis (rad)
%
% For rectangles:
%  10: length (m)
%  11: height (m)
%  12: orientation (rad) (relative to x, y already shown)
%
% For lines:
%  10: endpoint x-axis coordinate relative to start point (m)
%  11: endpoint y-axis coordinate relative to start point (m)
%
% For triangles:
%  10: length (m)
%  11: height (m)
%  12: offset of peak from midpoint of length (m)
%  13: orientation (rad)
%
% For all labelled target types:
%  14: reserved
%  15-64: label characters (indexes in ISO 8859-1 character set)
%  65: label colour (0xRRGGBB), opacity is set by the vcode's opacity (9).
%  66: label height (m)
%  67: reserved
%  68: reserved
%  69: reserved
%  70: reserved

num_targets = size(target, 1);

% NOTE: we assume that the STATE and/or OPACITY inputs are vectors. 

% If the length of the input STATE is not the same as the number of targets then make STATE a column vector of the same length as 
% the TARGET input, using the first STATE (i.e. all targets get the same state) 
if num_targets == length(state_in)
	state = reshape(state_in, num_targets, 1);
else
	state = state_in(1) * ones(num_targets, 1);
end


% If the length of the input OPACITY is not the same as the number of targets then make OPACITY a column vector of the same length as
% the TARGET input, using the first OPACITY (i.e. all targets get the same opacity) 
if num_targets == length(opacity_in)
	opacity = reshape(opacity_in, num_targets, 1);
else
	opacity = opacity_in(1) * ones(num_targets, 1);
end


% Clamping the opacity to [0, 100].
opacity = min(opacity, 100);
opacity = max(opacity, 0);

VCODE = zeros(num_targets, 70);

% Set the target type. Targets with labels have type codes 10 greater than their unlabelled counterparts.
VCODE(:, 1) = target_type + 10;

% Set the target position.
VCODE(:, 3) = target(:, x_index) * 0.01;  % x position (convert from (cm) in target table to (m))
VCODE(:, 4) = target(:, y_index) * 0.01;  % y position (convert from (cm) in target table to (m))

for ii = 1:num_targets
	% Set the target on/off state. If the state input is 0, the target is off. Users of the VCODE should respect this
	% as an indication that the rest of the VCODE will be uninitialized.
	if (state(ii) <= 0) || (state(ii) > num_states)
		VCODE(ii, 2) = 0;  % target is off
	else
		VCODE(ii, 2) = target_display;  % Default is that target is on; target displays as specified by block mask
	end

	fill_colour_col = stateindices(state(ii), 1);
	stroke_colour_col = stateindices(state(ii), 2);
	stroke_width_col = stateindices(state(ii), 3);
	
	% Set the fill colour. Fill colour currently comes from the GUI in RRRGGGBBB format.
	if fill_colour_col == 0
		VCODE(ii, 5) = -2^31;
	elseif target(fill_colour_col) < 0
		VCODE(ii, 5) = target(ii, fill_colour_col);
	else
		VCODE(ii, 5) = colourshift(target(ii, fill_colour_col));
	end
	
	% Set the stroke colour. Stroke colour currently comes from the GUI in RRRGGGBBB format.
	if stroke_colour_col == 0
		VCODE(ii, 6) = -2^31;
	elseif target(stroke_colour_col) < 0
		VCODE(ii, 6) = target(ii, stroke_colour_col);
	else
		VCODE(ii, 6) = colourshift( target(ii, stroke_colour_col) );
	end

	% Set the stroke width. if target table index for stroke width is zero, then the stroke width is undefined
	if stroke_width_col == 0
		VCODE(ii, 7) = 0;                   % if stroke width column is 0, then stroke width is 0
	elseif stroke_width_col < 0
		VCODE(ii, 7) = 0.001;               % if stroke width column is -ve, then a 1mm default is chosen
	else
		VCODE(ii, 7) = target(ii, stroke_width_col) * 0.01;  % if stroke width column is +ve, convert width from (cm) in target table to (m)
	end

	% Set the opacity value
	VCODE(ii, 9) = opacity(ii);

	% Set attributes specific to each target type. In the process, note the first state vector column used for label information.
	label_index = 1;

	% Set attributes specific to each target type.
	if target_type == 1

		% Handle circle target:
		radius_col = stateindices(state(ii), 4);
		VCODE(ii, 10)=target(ii, radius_col) * 0.01;  % radius (convert from (cm) in target table to (m))
	    label_index = 5;

	elseif target_type == 2 || target_type == 3

	    % Handle ellipse or rectangle target:
		major_col = stateindices(state(ii), 4);
		minor_col = stateindices(state(ii), 5);
		orientation_col = stateindices(state(ii), 6);
		
		VCODE(ii, 10) = target(ii, major_col) * 0.01;  % major radius (convert from (cm) in target table to (m))
		VCODE(ii, 11) = target(ii, minor_col) * 0.01;  % minor radius (convert from (cm) in target table to (m))
		if orientation_col == 0
			VCODE(ii, 12) = 0;  % if orientation column is 0, set orientation to 0 rad
		else
			VCODE(ii, 12) = mod(target(ii, orientation_col), 360) * pi / 180.0;  % orientation (convert from (degrees) in target table to (rad))
		end
	    label_index = 7;
	
	elseif target_type == 4

		% Handle line target:
		xendpoint_col = stateindices(state(ii), 4);
		yendpoint_col = stateindices(state(ii), 5);
		VCODE(ii, 10) = target(ii, xendpoint_col) * 0.01;  % line endpoint in x axis, relative to start (convert from (cm) in target table to (m))
		VCODE(ii, 11) = target(ii, yendpoint_col) * 0.01;  % line endpoint in y axis, relative to start (convert from (cm) in target table to (m))
	    label_index = 6;

	elseif target_type == 5

		% Handle triangle target:
		length_col = stateindices(state(ii), 4);
		height_col = stateindices(state(ii), 5);
		offset_col = stateindices(state(ii), 6);
		orientation_col = stateindices(state(ii), 7);

		VCODE(ii, 10) = target(ii, length_col) * 0.01;  % length (convert from (cm) in target table to (m))

		% If the height column is set to 0 then the triangle is automatically made equilateral, with the base length used as length
		% for all sides. If the height column is non-zero, separate values for height and peak offset are taken from the target table.
		if height_col == 0
			VCODE(ii, 11) = sin(pi / 3.0) * VCODE(ii, 10);  % height for equilateral triangle
			VCODE(ii, 12) = 0;                          % peak offset for equilateral triangle
		else
			VCODE(ii, 11) = target(ii, height_col) * 0.01;  % height (convert from (cm) in target table to (m))
			VCODE(ii, 12) = target(ii, offset_col) * 0.01;  % peak offset (convert from (cm) in target table to (m))
		end

		if orientation_col == 0
			VCODE(ii, 13) = 0;  % if orientation column is 0, set orientation to 0 rad
		else
			VCODE(ii, 13) = mod(target(ii, orientation_col), 360) * pi / 180.0;  % orientation (convert from (degrees) in target table to (rad))
		end
	    label_index = 8;
		
	end
	
	% Copy the label characters to the VCODE.
	for jj = 1:50
		VCODE(ii, jj + 14) = target_labels( target( ii, stateindices(state(ii), label_index) ), jj );
	end

	% Set the label colour. Like other colours, label colour comes from the GUI in RRRGGGBBB format and is converted to a 32-bit
	% 0xRRGGBB value here. If the target column table index for the colour is 0, the label is transparent.
	if stateindices(state(ii), label_index + 1) == 0
		VCODE(ii, 65) = -2^31;
	elseif target( ii, stateindices(state(ii), label_index + 1) ) < 0
		VCODE(ii, 65) = target( ii, stateindices(state(ii), label_index + 1) );
	else
		VCODE(ii, 65) = colourshift( target( ii, stateindices(state(ii), label_index + 1) ) );
	end

	% Set the label height. Label height is converted from (cm) in the target table to (m).
	VCODE(ii, 66) = target( ii, stateindices(state, label_index + 2) ) * 0.01;


	
end

% The colourshift function converts an "RRRGGGBBB" colour value to RRGBB (as an uint32).
function RRGGBBAA = colourshift(RRRGGGBBB)

%this is "no fill"
if RRRGGGBBB == 1000000000
    RRGGBBAA = cast(16777216, 'uint32'); %hex 0x1000000
    return; 
end

blue = cast(mod(RRRGGGBBB, 1000), 'uint32');
green = cast(mod(RRRGGGBBB - blue, 1000000) / 1000, 'uint32');
red = cast((RRRGGGBBB - (green * 1000) - blue) / 1000000, 'uint32');

RRGGBBAA = bitshift(red, 16) + bitshift(green, 8) + blue;
%}
